simulink model "lab_02_model"  (R2021a)
settings: Solver=VariableStepAuto  StartTime=0.0  StopTime=0.05  RelTol=1e-3
libraries: spsThreePhaseSeriesRLCBranchLib x2, spsThreePhaseTransformerTwoWindingsLib x2, spsGroundLib x1, spsMultimeterLib x1, spsThreePhaseVIMeasurementLib x1, spsThreePhaseSourceLib x1, spspowerguiLib x1
settings Model: Creator=muham  LastModifiedBy=muham
settings DebuggingCC: UnconnectedInputMsg=none  UnconnectedOutputMsg=none  UnconnectedLineMsg=none

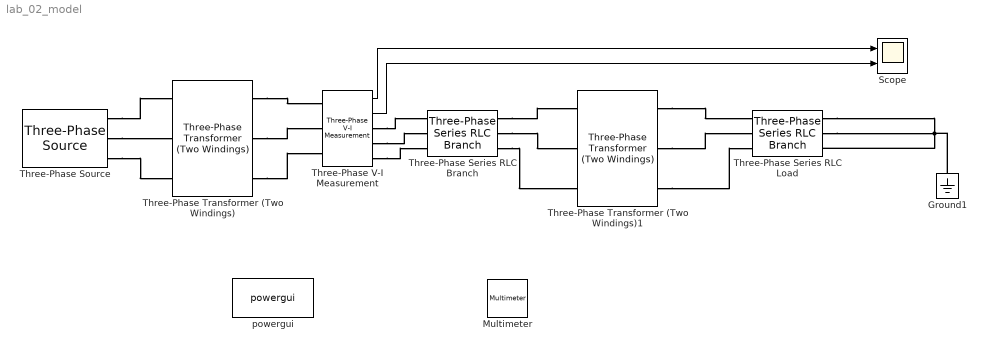
== system lab_02_model ==
  Ground1 : spsGroundLib/Ground  LConnTagsString=a
  Multimeter : spsMultimeterLib/Multimeter  PhasorSimulation=off  OutputType=Complex  sel=[8 10 13 16 21 21 21 21 21 21 21 21 21 21 21 21 21 21 21 21]  L=54  Gain=[1 1 1 1 1 1 1 1 1 1 1 1 1 1 1 1 1 1 1 1]  yselected={'Ubg_w1: Three-Phase Transformer (Two Windings)','Uag_w2: Three-Phase Transformer (Two Windings)','Uag_w1: Three-Phase Transformer (Two Windings)1','Uag_w2: Three-Phase Transformer (Two Windings)1','Ib3: Three-Phase Series RLC Branch','Ib3: Three-Phase Series RLC Branch','Ib3: Three-Phase Series RLC Branch','Ib3: Three-Phase Series RLC Branch','Ib3: Three-Phase Series RLC Branch','Ib3: Three-Phase Series RLC Branch','Ib3: Three-Phase Series RLC Branch','Ib3: Three-Phase Series RLC Branch','Ib3: Three-Phase Series RLC Branch','Ib3: Three-Phase Series RLC Branch','Ib3: Three-Phase Series RLC Branch','Ib3: Three-Phase Series RLC Branch','Ib3: Three-Phase Series RLC Branch','Ib3: Three-Phase Series RLC Branch','Ib3: Three-Phase Series RLC Branch','Ib3: Three-Phase Series RLC Branch'};  PSBOutputType=1  PSBequivalent=0  AxesSetting=[0,0.1,-100,100]  Display=1  SavedBlockNames=-11
  Scope : Scope  NumInputPorts=2
  Three-Phase Series RLC Branch : spsThreePhaseSeriesRLCBranchLib/Three-Phase Series RLC Branch  LConnTagsString=A|B|C  RConnTagsString=A|B|C  BranchType=L  Resistance=0  Inductance=20/(2*pi*60)  Capacitance=inf  Measurements=Branch voltages and currents
  Three-Phase Series RLC Load : spsThreePhaseSeriesRLCBranchLib/Three-Phase Series RLC Branch  LConnTagsString=A|B|C  RConnTagsString=A|B|C  BranchType=RLC  Resistance=0.64  Inductance=0.48/(2*pi*60)  Capacitance=inf  Measurements=Branch voltages and currents
  Three-Phase Transformer (Two Windings) : spsThreePhaseTransformerTwoWindingsLib/Three-Phase Transformer (Two Windings)  Winding1Connection=Yg  Winding2Connection=Yg  CoreType=Three single-phase transformers  SetSaturation=off  Hysteresis=off  DataFile='hysteresis'  SetInitialFlux=off  Measurements=All measurements (V I Fluxes)  UNITS=pu  NominalPower=[ 150e6 , 50 ]  Winding1=[ 13.8e3 , 0 , 0.1]  Winding2=[ 138e3 , 0 , 0 ]  Rm=500  Lm=500  L0=0.5  Saturation=[ 0,0 ; 0.0024,1.2 ; 1.0,1.52 ]  InitialFluxes=[ 0.8 , -0.8 , 0.7 ]  BreakLoop=off  DiscreteSolver=Trapezoidal iterative  DataType=off  TransfoNumber=1
  Three-Phase Transformer (Two Windings)1 : spsThreePhaseTransformerTwoWindingsLib/Three-Phase Transformer (Two Windings)  Winding1Connection=Yg  Winding2Connection=Yg  CoreType=Three single-phase transformers  SetSaturation=off  Hysteresis=off  DataFile='hysteresis'  SetInitialFlux=off  Measurements=All measurements (V I Fluxes)  UNITS=pu  NominalPower=[ 125e6 , 50 ]  Winding1=[132e3 0 0.1]  Winding2=[11e3 0 0]  Rm=500  Lm=500  L0=0.5  Saturation=[0 0;0.0024 1.2;1 1.52]  InitialFluxes=[ 0.8 , -0.8 , 0.7 ]  BreakLoop=off  DiscreteSolver=Trapezoidal iterative  DataType=off  TransfoNumber=1
  Three-Phase V-I Measurement : spsThreePhaseVIMeasurementLib/Three-Phase V-I Measurement  VoltageMeasurement=phase-to-ground  SetLabelV=off  LabelV=Vabc  Vpu=off  VpuLL=off  CurrentMeasurement=yes  SetLabelI=off  LabelI=Iabc  Ipu=off  Pbase=100e6  Vbase=500e3  OutputType=Complex  PhasorSimulation=off  PSBequivalent=0
  Three-Phase Source : spsThreePhaseSourceLib/Three-Phase Source  InternalConnection=Yg  VoltagePhases=off  Voltage=13.2e3  PhaseAngle=0  Voltage_phases=[25e3 25e3 25e3]/sqrt(3)  PhaseAngles_phases=[0 -120 +120]  Frequency=50  NonIdealSource=on  SpecifyImpedance=off  Resistance=0  Inductance=0.4/(2*pi*60)  ShortCircuitLevel=100e6  BaseVoltage=25e3  XRratio=7  BusType=swing  Pref=10e3  Qref=0  Prefabc=[10e3, 10e3, 10e3]  Qrefabc=[0, 0, 0]  Qmin=-inf  Qmax=inf
  powergui : spspowerguiLib/powergui  Priority=1  SimulationMode=Continuous  SampleTime=50e-6  frequency=60  Iterations=50  frequencyindice=50  Pbase=100e6  ErrMax=1e-4  UnitsV=kV  UnitsW=MW  buscounter=0  FunctionMessages=off  echomessages=off  EnableUseOfTLC=off  CurrentSourceSwitches=off  DisableSnubberDevices=off  DisableRonSwitches=off  DisableVfSwitches=off  DisplayEquations=off  AutomaticDiscreteSolvers=off  SolverType=Tustin/Backward Euler (TBE)  Interpol=off  ExternalGateDelay=off  methode=off  Ts=100  x0status=blocks  SPID=on  SwTol=0  HookPort=off  NonlinearTolerance=1e-4  nMaxIteration=100  ContinueOnMaxIteration=off  RestoreLinks=warning  ResistiveCurrentMeasurement=off  Frange=[0:2:500]  Ylog=off  Xlog=on  ShowGrid=off  save=off  variable=ZData  structure=0  ZoomFFT=off  StartTime=0.0  cycles=1  DisplayStyle=1  fundamental=60  FreqAxis=off  MaxFrequency=1000  frequencyindicesteady=1  RmsSteady=1  display=off
  wires:
  Three-Phase V-I Measurement/1 -> Scope/1
  Three-Phase V-I Measurement/2 -> Scope/2
  connections:
  Three-Phase Source/RConn1 -- Three-Phase Transformer (Two Windings)/LConn1
  Three-Phase Source/RConn2 -- Three-Phase Transformer (Two Windings)/LConn2
  Three-Phase Source/RConn3 -- Three-Phase Transformer (Two Windings)/LConn3
  Three-Phase Transformer (Two Windings)/RConn1 -- Three-Phase V-I Measurement/LConn1
  Three-Phase Transformer (Two Windings)/RConn2 -- Three-Phase V-I Measurement/LConn2
  Three-Phase Transformer (Two Windings)/RConn3 -- Three-Phase V-I Measurement/LConn3
  Three-Phase Series RLC Load/RConn1 -- Three-Phase Series RLC Load/RConn2 -- Ground1/LConn1 -- Three-Phase Series RLC Load/RConn3
  Three-Phase V-I Measurement/RConn1 -- Three-Phase Series RLC Branch/LConn1
  Three-Phase V-I Measurement/RConn2 -- Three-Phase Series RLC Branch/LConn2
  Three-Phase V-I Measurement/RConn3 -- Three-Phase Series RLC Branch/LConn3
  Three-Phase Series RLC Branch/RConn1 -- Three-Phase Transformer (Two Windings)1/LConn1
  Three-Phase Series RLC Branch/RConn2 -- Three-Phase Transformer (Two Windings)1/LConn2
  Three-Phase Series RLC Branch/RConn3 -- Three-Phase Transformer (Two Windings)1/LConn3
  Three-Phase Transformer (Two Windings)1/RConn1 -- Three-Phase Series RLC Load/LConn1
  Three-Phase Transformer (Two Windings)1/RConn2 -- Three-Phase Series RLC Load/LConn2
  Three-Phase Transformer (Two Windings)1/RConn3 -- Three-Phase Series RLC Load/LConn3
